simulink model "acf_sea_pad_research_20261006"  (R2026b)
settings: Solver=ode4  StopTime=p.stopTime  FixedStep=2.5000000000000002e-06
model workspace (MAT data in the model file):
  p.dt = 2.5e-06
  p.controlStep = 0.0001
  p.stopTime = 2
  p.mA = 1.5
  p.mB = 0.6
  p.mS = 1.4
  p.gAxis = 6.93434871572
  p.Fref = 20
  p.kUpper = 20000
  p.kCell = 64000000
  p.sea = 0
  p.mNut = 0.075
  p.kSea = 5000
  p.cSea = 0
  p.preload = 0
  p.ell = 0.00159154943092
  p.Jtotal = 7.04e-06
  p.Kf = 24.4
  p.Kt = 0.0758
  p.Ke = 0.0758
  p.R = 8.896
  p.L = 0.004
  p.Imax = 3.5
  p.Vmax = 32
  p.currentTau = 5e-05
  p.guideCoulomb = 0.2
  p.guideViscous = 2
  p.guideSmooth = 0.001
  p.shaftCoulomb = 0.001
  p.shaftViscous = 1e-06
  p.shaftSmooth = 1
  p.kPad = 20000
  p.cPad = 80
  p.padDiameter = 0
  p.stripCount = 61
  p.bumpTime = 0.8
  p.bumpHeight = 0.001
  p.bumpWidth = 0.01
  p.scanSpeed = 0.1
  p.toolTravelLimit = 0.0125
  p.nutTravelLimit = 0.05
  p.springTravelLimit = 0.017
  p.padCompressionLimit = 0.005
  p.enableStops = 1
  p.offsets = 0
  p.weights = 1
  p.centerWeight = 1
  p.rigidPoint = 0
  p.initial = [-0.000213511025252 0 -0.00100016081112 0 -0.001 0 0 0 0.251282892154]
  p.massInverse = [0.635716076883  0.0167042812039; 0.0167042812039  0.350789905281]
  replayInputs = [0 0.0001 0.0002 0.0003 0.0004 0.0005 0.0006 0.0007 0.0008 0.0009 0.001 0.0011 ... (60003 elements, 20001x3)]
libraries: simulink x1
(part 1 of 2)
settings Model: Creator=tommie  LastModifiedBy=tommie
settings DataIOCC: ExternalInput=replayInputs  LoadExternalInput=on  SignalLogging=off

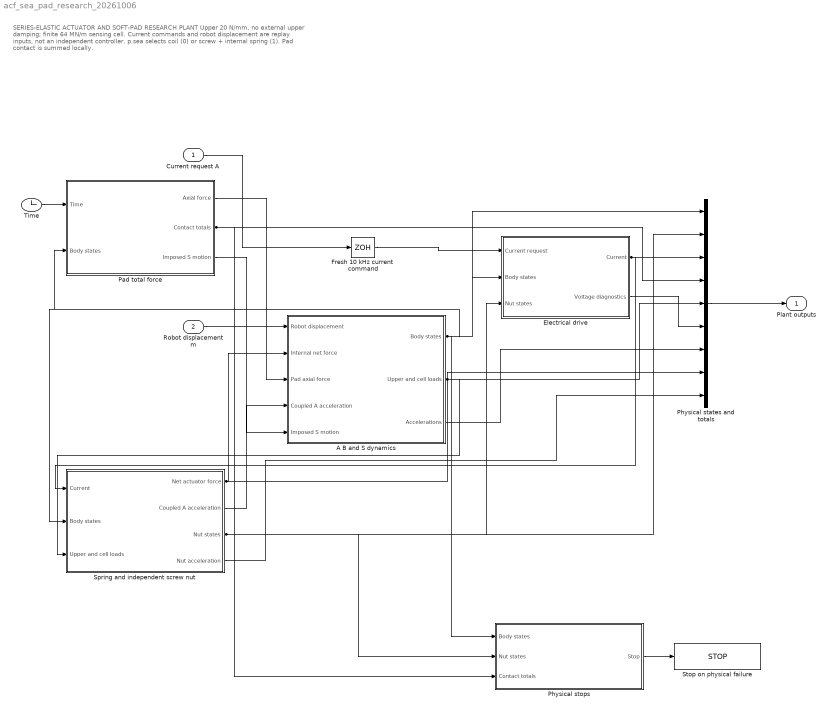
== system acf_sea_pad_research_20261006 ==
  note: SERIES-ELASTIC ACTUATOR AND SOFT-PAD RESEARCH PLANT
      | Upper 20 N/mm, no external upper damping; finite 64 MN/m sensing cell.
      | Current commands and robot displacement are replay inputs, not an independent controller.
      | p.sea selects coil (0) or screw + internal spring (1). Pad contact is summed locally.
  Current request A : Inport
  Robot displacement m : Inport  Port=2
  A B and S dynamics : Subsystem
  Electrical drive : Subsystem
  Fresh 10 kHz current command : ZeroOrderHold  SampleTime=p.controlStep
  Pad total force : Subsystem
  Physical states and totals : Mux  Inputs=9
  Physical stops : Subsystem
  Spring and independent screw nut : Subsystem
  Stop on physical failure : Stop
  Time : Clock
  Plant outputs : Outport
  wires:
  Physical stops/1(Stop) -> Stop on physical failure/1
  Electrical drive/2(Voltage diagnostics) -> Physical states and totals/6
  Electrical drive/1(Current) -> Physical states and totals/3, Spring and independent screw nut/1(Current)
  Physical states and totals/1 -> Plant outputs/1
  A B and S dynamics/3(Accelerations) -> Physical states and totals/7
  Current request A/1 -> Fresh 10 kHz current command/1
  Time/1 -> Pad total force/1(Time)
  Spring and independent screw nut/2(Coupled A acceleration) -> A B and S dynamics/4(Coupled A acceleration)
  Pad total force/1(Axial force) -> A B and S dynamics/3(Pad axial force)
  Pad total force/2(Contact totals) -> Physical stops/3(Contact totals), Physical states and totals/4
  Pad total force/3(Imposed S motion) -> A B and S dynamics/5(Imposed S motion)
  Spring and independent screw nut/1(Net actuator force) -> A B and S dynamics/2(Internal net force), Physical states and totals/8
  Spring and independent screw nut/3(Nut states) -> Physical states and totals/2, Physical stops/2(Nut states), Electrical drive/3(Nut states)
  Robot displacement m/1 -> A B and S dynamics/1(Robot displacement)
  Fresh 10 kHz current command/1 -> Electrical drive/1(Current request)
  Spring and independent screw nut/4(Nut acceleration) -> Physical states and totals/9
  A B and S dynamics/1(Body states) -> Physical stops/1(Body states), Electrical drive/2(Body states), Physical states and totals/1, Pad total force/2(Body states), Spring and independent screw nut/2(Body states)
  A B and S dynamics/2(Upper and cell loads) -> Physical states and totals/5, Spring and independent screw nut/3(Upper and cell loads)
